simulink model "bess_resource_standalone"  (R2023b)
settings: Solver=ode23t  StartTime=0.0  StopTime=0.8  MaxStep=1e-5  RelTol=1e-3
InitFcn:
  | root=fileparts(fileparts(fileparts(get_param(bdroot,'FileName')))); addpath(root); setup_v2_paths; define_resource_buses(true); define_v2_parameters(true);
undefined symbols (not defined in the file): V2
libraries: ee_lib x12, nesl_utility x9, simulink x3, fl_lib x1
settings Model: Creator=fakebob2004  LastModifiedBy=fakebob2004
settings ModelReferenceCC: UpdateModelReferenceTargets=IfOutOfDate
settings RTWCC: GPUComputeCapability=5.0
settings ConfigComp: CovBoundaryAbsTol=1.0e-5
settings SimscapeCC: SimscapeNominalValues="[{\"value\":\"1\",\"unit\":\"A\"},{\"value\":\"1\",\"unit\":\"bar\"},{\"value\":\"1\",\"unit\":\"cm^2\"},{\"value\":\"1\",\"unit\":\"cm^3/s\"},{\"value\":\"1\",\"unit\":\"kJ/kg\"},{\"value\":\"1\",\"unit\":\"kW\"},{\"value\":\"1\",\"unit\":\"l\"},{\"value\":\"1\",\"unit\":\"N\"},{\"value\":\"1\",\"unit\":\"N*m\"},{\"value\":\"1\",\"unit\":\"V\"},{\"value\":\"0.001\",\"unit\":\"Wb\"}]"  SimscapeLogType=all  SimscapeLogDataHistory=10000

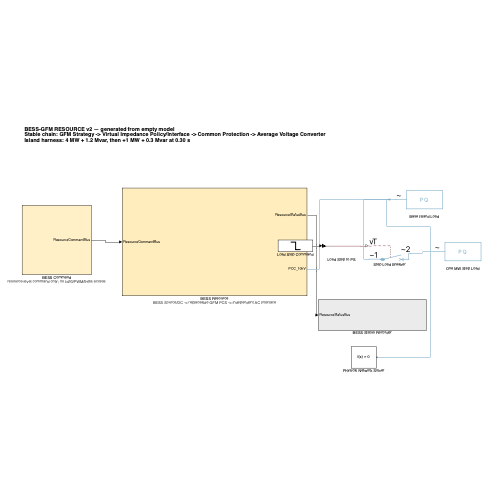
[thumbnail: Simulink's stored preview of the top-level diagram]
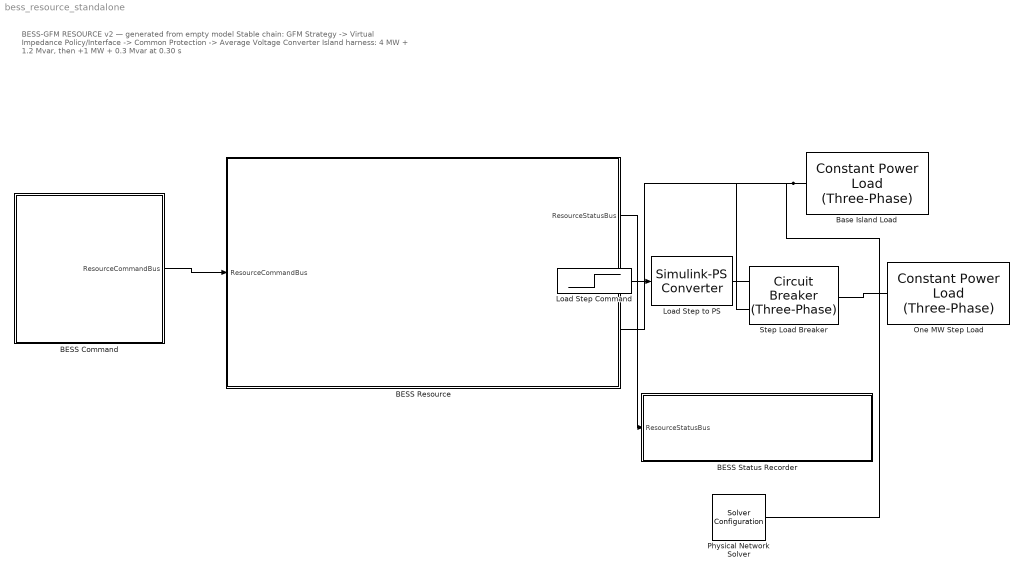
== system bess_resource_standalone ==
  note: BESS-GFM RESOURCE v2 — generated from empty model
      | Stable chain: GFM Strategy -> Virtual Impedance Policy/Interface -> Common Protection -> Average Voltage Converter
      | Island harness: 4 MW + 1.2 Mvar, then +1 MW + 0.3 Mvar at 0.30 s
  BESS Command : Subsystem
      settings: AttributesFormatString=resource-level command only; no Id/Iq/PWM/theta access
  BESS Resource : Subsystem
      settings: AttributesFormatString=BESS Source/DC -> replaceable GFM PCS -> independent AC Interface
  BESS Status Recorder : Subsystem
  Base Island Load : ee_lib/Passive/Constant Power Load (Three-Phase)  port_option=ee.enum.threePhasePort.composite  FRated=V2.BESS.rating.f_Hz Hz  active_power=4e6 W  reactive_power=1.2e6 V*A  Vline_rms_min=0.70*V2.BESS.rating.V_pcc_V V  tau=0.01 s  Vline_rms_ini=V2.BESS.rating.V_pcc_V V  Vang_ini=0 deg  gmin=1e-6 S
  Load Step Command : Step  Time=.30  Before=1  After=0  SampleTime=0
  Load Step to PS : nesl_utility/Simulink-PS Converter  PhysicalDomain=network_engine_domain  SubClassName=ps_input  LeftPortType=input  RightPortType=output  PseudoPeriodic=off  Frequencies=[]  NoiseDistribution=none  NoiseParameters=[]  Unit=V  AffineConversion=off  FilteringAndDerivatives=zero  SimscapeFilterOrder=1  InputFilterTimeConstant=0.001  UdotUserProvided=0
  One MW Step Load : ee_lib/Passive/Constant Power Load (Three-Phase)  port_option=ee.enum.threePhasePort.composite  FRated=V2.BESS.rating.f_Hz Hz  active_power=1e6 W  reactive_power=0.3e6 V*A  Vline_rms_min=0.70*V2.BESS.rating.V_pcc_V V  tau=0.01 s  Vline_rms_ini=V2.BESS.rating.V_pcc_V V  Vang_ini=0 deg  gmin=1e-6 S
  Physical Network Solver : nesl_utility/Solver Configuration  PhysicalDomain=network_engine_domain  SubClassName=solver  LeftPortType=input  RightPortType=generic  Tones=[]  Harmonics=[]  SimulateNoise=off  Profile=off  UseLocalSampling=off  EnableSwitchedLinearOptims=on  FrequencyDomain=off  UseCCode=off  RelTol=0.001  AbsTol=0.001  MinStep=1e-09  ToWorkspace=off  RevertToSquareIcSolve=off  NumHomotopyIterations=100  PhasorMode=off  PhasorModeNumHarmonics=1  ConsistencySolver=NEWTON_XTOL_AFTER_FTOL  CanonicalOrdering=CANONICAL  OptimizeIntermediates=OPTIMIZED  IndexReductionMethod=DerivativeReplacement  DoDC=off  ResidualTolerance=1e-09  ConsistencyTolSource=GLOBAL  ConsistencyAbsTol=0.001  ConsistencyRelTol=0.001  ConsistencyTolFactor=0.001  UseLocalSolver=off  LocalSolverChoice=NE_BACKWARD_EULER_ADVANCER  ResolveIndetEquations=on  FunctionEvalNumThread=1  LocalSolverSampleTime=0.001  DoFixedCost=off  MaxNonlinIter=3  MaxModeIter=2  ComputeImpulses=off  ImpulseIterations=2  LinearAlgebra=auto  LinearAlgebraNumThread=0  EquationFormulation=NE_TIME_EF  DelaysMemoryBudget=1024  AutomaticFiltering=on  FilteringTimeConstant=0.001  PartitionStorageMethod=AS_NEEDED  PartitionMemoryBudget=1024  PartitionMethod=ROBUST  MultibodyUseLocalSolver=off  MultibodyLocalSolverChoice=ODE1  MultibodyLocalSolverSampleTime=0.001
  Step Load Breaker : ee_lib/Switches & Breakers/Circuit Breaker (Three-Phase)  port_option=ee.enum.threePhasePort.composite  control_port_option=ee.enum.controlport.ps  R_closed=0.001 Ohm  G_open=1e-6 1/Ohm  threshold=0.5 V  breaker_behavior=ee.enum.switches.breakerBehavior.zeroCrossingEnable  i_th=1e-8 A
  wires:
  Load Step Command/1 -> Load Step to PS/1
  BESS Command/1(ResourceCommandBus) -> BESS Resource/1(ResourceCommandBus)
  BESS Resource/1(ResourceStatusBus) -> BESS Status Recorder/1(ResourceStatusBus)
  connections:
  Base Island Load/LConn1 -- BESS Resource/RConn1 -- Step Load Breaker/LConn2 -- Physical Network Solver/RConn1
  Step Load Breaker/RConn1 -- One MW Step Load/LConn1
  Load Step to PS/RConn1 -- Step Load Breaker/LConn1

== system bess_resource_standalone/BESS Command ==
  Enable : Constant
  Mode : Constant
  P ref : Constant  Value=4e6
  Q ref : Constant  Value=1.2e6
  Resource Command : BusCreator  Inputs=6  OutDataTypeStr=Bus: ResourceCommandBus
  V ref : Constant  Value=690
  f ref : Constant  Value=50
  ResourceCommandBus : Outport  OutDataTypeStr=Bus: ResourceCommandBus
  wires:
  P ref/1 -> Resource Command/1  "P_ref_W"
  Q ref/1 -> Resource Command/2  "Q_ref_var"
  V ref/1 -> Resource Command/3  "V_ref_V"
  f ref/1 -> Resource Command/4  "f_ref_Hz"
  Enable/1 -> Resource Command/5  "enable"
  Mode/1 -> Resource Command/6  "mode"
  Resource Command/1 -> ResourceCommandBus/1

== system bess_resource_standalone/BESS Resource ==
  ResourceCommandBus : Inport  OutDataTypeStr=Bus: ResourceCommandBus
  01 BESS Source and DC Side : Subsystem
      settings: AttributesFormatString=5 MW / 10 MWh | replaceable energy model -> local limits/status
  02 PCS : Subsystem
      settings: AttributesFormatString=strategy slot -> VI policy/interface -> common protection -> average voltage source
  03 AC Interface : Subsystem
      settings: AttributesFormatString=independent filter + 0.69/10 kV transformer + PCC sensing
  Status Interface : Subsystem
      settings: AttributesFormatString=BESS + GFM PCS + PCC -> ResourceStatusBus
  PCC_10kV : PMIOPort  Side=Right  ConnectionType=Connection: foundation.electrical.three_phase
  ResourceStatusBus : Outport  OutDataTypeStr=Bus: ResourceStatusBus
  wires:
  ResourceCommandBus/1 -> 02 PCS/1(CommandBus)
  03 AC Interface/1(PCCMeasurementBus) -> 01 BESS Source and DC Side/1(PCCMeasurementBus), 02 PCS/2(PCCMeasurementBus), Status Interface/3(PCC)
  01 BESS Source and DC Side/1(BESSStatusBus) -> 02 PCS/3(BESSStatusBus)
  01 BESS Source and DC Side/2(SourceStatusBus) -> Status Interface/1(Source)
  02 PCS/1(GFMPCSStatusBus) -> Status Interface/2(PCS)
  Status Interface/1(ResourceStatusBus) -> ResourceStatusBus/1
  connections:
  02 PCS/RConn1 -- 03 AC Interface/LConn1
  03 AC Interface/RConn1 -- PCC_10kV/RConn1

== system bess_resource_standalone/BESS Status Recorder ==
  ResourceStatusBus : Inport  OutDataTypeStr=Bus: ResourceStatusBus
  BESS v2 Result : ToWorkspace  VariableName=bess_v2_result  SampleTime=-1
  Regression Vector : Mux  Inputs=12
  Status Selector : BusSelector  OutputSignals=P_W,Q_var,Vpcc_V,frequency_Hz,available_power_W,power_headroom_W,current_limit_factor,energy_state_pu,Vdc_V,control_mode,healthy
  Time : Clock
  wires:
  Time/1 -> Regression Vector/1
  Status Selector/1 -> Regression Vector/2  "<P_W>"
  Status Selector/2 -> Regression Vector/3  "<Q_var>"
  Status Selector/3 -> Regression Vector/4  "<Vpcc_V>"
  Status Selector/4 -> Regression Vector/5  "<frequency_Hz>"
  Status Selector/5 -> Regression Vector/6  "<available_power_W>"
  Status Selector/6 -> Regression Vector/7  "<power_headroom_W>"
  Status Selector/7 -> Regression Vector/8  "<current_limit_factor>"
  Status Selector/8 -> Regression Vector/9  "<energy_state_pu>"
  Status Selector/9 -> Regression Vector/10  "<Vdc_V>"
  Status Selector/10 -> Regression Vector/11  "<control_mode>"
  Status Selector/11 -> Regression Vector/12  "<healthy>"
  ResourceStatusBus/1 -> Status Selector/1
  Regression Vector/1 -> BESS v2 Result/1

== system bess_resource_standalone/BESS Resource/01 BESS Source and DC Side ==
  PCCMeasurementBus : Inport  OutDataTypeStr=Bus: PCCMeasurementBus
  01 Energy and DC State : Subsystem
      settings: AttributesFormatString=PCC P -> DC buffer/loss -> SOC, Vdc, Ibat
  02 Limits and Availability : Subsystem
      settings: AttributesFormatString=SOC direction + Ibat limit -> common resource status
  BESSStatusBus : Outport  OutDataTypeStr=Bus: BESSStatusBus
  SourceStatusBus : Outport  Port=2  OutDataTypeStr=Bus: SourceStatusBus
  wires:
  PCCMeasurementBus/1 -> 01 Energy and DC State/1(PCCMeasurementBus)
  01 Energy and DC State/1(BESSDCStateBus) -> 02 Limits and Availability/1(BESSDCStateBus)
  02 Limits and Availability/1(BESSStatusBus) -> BESSStatusBus/1
  02 Limits and Availability/2(SourceStatusBus) -> SourceStatusBus/1

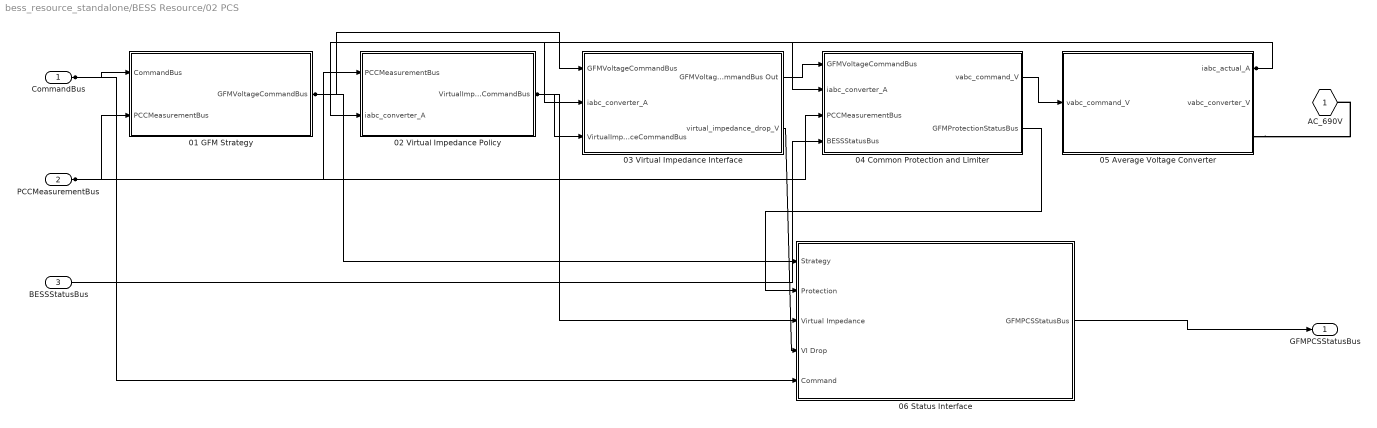
== system bess_resource_standalone/BESS Resource/02 PCS ==
  CommandBus : Inport  OutDataTypeStr=Bus: ResourceCommandBus
  PCCMeasurementBus : Inport  Port=2  OutDataTypeStr=Bus: PCCMeasurementBus
  BESSStatusBus : Inport  Port=3  OutDataTypeStr=Bus: BESSStatusBus
  01 GFM Strategy : Subsystem
      settings: AttributesFormatString=replaceable P-f/Q-V strategy -> typed voltage command
  02 Virtual Impedance Policy : Subsystem
      settings: AttributesFormatString=replaceable static/dynamic VI policy -> enable, R, X
  03 Virtual Impedance Interface : Subsystem
      settings: AttributesFormatString=current conditioning -> R+jX drop -> compensated voltage command
  04 Common Protection and Limiter : Subsystem
      settings: AttributesFormatString=strategy-independent voltage/SOC/current backup protection
  05 Average Voltage Converter : Subsystem
  06 Status Interface : Subsystem
      settings: AttributesFormatString=strategy + VI + protection -> GFMPCSStatusBus
  AC_690V : PMIOPort  Side=Right  ConnectionType=Connection: foundation.electrical.three_phase
  GFMPCSStatusBus : Outport  OutDataTypeStr=Bus: GFMPCSStatusBus
  wires:
  CommandBus/1 -> 01 GFM Strategy/1(CommandBus), 06 Status Interface/5(Command)
  PCCMeasurementBus/1 -> 01 GFM Strategy/2(PCCMeasurementBus), 02 Virtual Impedance Policy/1(PCCMeasurementBus), 04 Common Protection and Limiter/3(PCCMeasurementBus)
  05 Average Voltage Converter/1(iabc_actual_A) -> 02 Virtual Impedance Policy/2(iabc_converter_A), 03 Virtual Impedance Interface/2(iabc_converter_A), 04 Common Protection and Limiter/2(iabc_converter_A)
  01 GFM Strategy/1(GFMVoltageCommandBus) -> 03 Virtual Impedance Interface/1(GFMVoltageCommandBus), 06 Status Interface/1(Strategy)
  02 Virtual Impedance Policy/1(VirtualImpedanceCommandBus) -> 03 Virtual Impedance Interface/3(VirtualImpedanceCommandBus), 06 Status Interface/3(Virtual Impedance)
  03 Virtual Impedance Interface/1(GFMVoltageCommandBus Out) -> 04 Common Protection and Limiter/1(GFMVoltageCommandBus)
  BESSStatusBus/1 -> 04 Common Protection and Limiter/4(BESSStatusBus)
  04 Common Protection and Limiter/1(vabc_command_V) -> 05 Average Voltage Converter/1(vabc_command_V)
  04 Common Protection and Limiter/2(GFMProtectionStatusBus) -> 06 Status Interface/2(Protection)
  03 Virtual Impedance Interface/2(virtual_impedance_drop_V) -> 06 Status Interface/4(VI Drop)
  06 Status Interface/1(GFMPCSStatusBus) -> GFMPCSStatusBus/1
  connections:
  05 Average Voltage Converter/RConn1 -- AC_690V/RConn1

== system bess_resource_standalone/BESS Resource/03 AC Interface ==
  Damped Shunt C : ee_lib/Passive/RLC Assemblies/RLC (Three-Phase)  port_option=ee.enum.threePhasePort.composite  component_structure=ee.enum.rlc.structure.SeriesRC  R=V2.BESS.filter.Rd_ohm Ohm  L=1e-3 H  C=V2.BESS.filter.C_F F  R_parasitic=0 Ohm  G_parasitic=0 1/Ohm  IL_specify=off  IL_priority=High  IL=[0, 0, 0] A  IL_nominal_specify=off  IL_nominal_value=1  IL_nominal_unit=A  VC_specify=off  VC_priority=High  VC=[0, 0, 0] V  VC_nominal_specify=off  VC_nominal_value=1  VC_nominal_unit=V
  Filter Ground : ee_lib/Connectors & References/Grounded Neutral (Three-Phase)  port_option=ee.enum.threePhasePort.composite
  Grid-side R2 + L2 : ee_lib/Passive/RLC Assemblies/RLC (Three-Phase)  port_option=ee.enum.threePhasePort.composite  component_structure=ee.enum.rlc.structure.SeriesRL  R=V2.BESS.filter.R2_ohm Ohm  L=V2.BESS.filter.L2_H H  C=1e-6 F  R_parasitic=0 Ohm  G_parasitic=0 1/Ohm  IL_specify=off  IL_priority=High  IL=[0, 0, 0] A  IL_nominal_specify=off  IL_nominal_value=1  IL_nominal_unit=A  VC_specify=off  VC_priority=High  VC=[0, 0, 0] V  VC_nominal_specify=off  VC_nominal_value=1  VC_nominal_unit=V
  Inverter-side R1 + L1 : ee_lib/Passive/RLC Assemblies/RLC (Three-Phase)  port_option=ee.enum.threePhasePort.composite  component_structure=ee.enum.rlc.structure.SeriesRL  R=V2.BESS.filter.R1_ohm Ohm  L=V2.BESS.filter.L1_H H  C=1e-6 F  R_parasitic=0 Ohm  G_parasitic=0 1/Ohm  IL_specify=off  IL_priority=High  IL=[0, 0, 0] A  IL_nominal_specify=off  IL_nominal_value=1  IL_nominal_unit=A  VC_specify=off  VC_priority=High  VC=[0, 0, 0] V  VC_nominal_specify=off  VC_nominal_value=1  VC_nominal_unit=V
  PCC Measurement : Subsystem
  Step-up Transformer : ee_lib/Passive/Transformers/Two-Winding Transformer (Three-Phase)  SRated=V2.BESS.transformer.S_VA A*V  FRated=V2.BESS.rating.f_Hz Hz  Winding1Connection=ee.enum.windingconnection.Yg  VRated1=V2.BESS.transformer.V1_V V  Winding2Connection=ee.enum.windingconnection.Yg  VRated2=V2.BESS.transformer.V2_V V  CoreType=ee.enum.coretype.threelimb  pu_Rw1=V2.BESS.transformer.R_pu/2  pu_Rw2=V2.BESS.transformer.R_pu/2  leakage_reactance_option=ee.enum.transformer_leakage.exclude  pu_Xl1=0.05  pu_Xl2=0.05  magnetizing_resistance_option=ee.enum.transformer_magnetizingResistance.exclude  pu_Rm=500  magnetizing_reactance_option=ee.enum.transformer_magnetizingReactance.exclude  saturation_option=ee.enum.transformer_saturation.exclude  pu_Xm=500  current_data=[0, .002, 1, 2]  magnetic_flux_data=[0, 1.2, 1.5, 1.51]  pu_X0=0.5  i1_specify=off  i1_priority=None  i1=[0, 0, 0] A  i1_nominal_specify=off  i1_nominal_value=1  i1_nominal_unit=A  i2_specify=off  i2_priority=None  i2=[0, 0, 0] A  i2_nominal_specify=off  i2_nominal_value=1  i2_nominal_unit=A  phi_specify=off  phi_priority=None  phi=[0, 0, 0]  phi_nominal_specify=off  phi_nominal_value=1  phi_nominal_unit=1
  PCS AC Terminal : PMIOPort  Side=Left  ConnectionType=Connection: foundation.electrical.three_phase
  PCC_10kV : PMIOPort  Port=2  Side=Right  ConnectionType=Connection: foundation.electrical.three_phase
  PCCMeasurementBus : Outport  OutDataTypeStr=Bus: PCCMeasurementBus
  wires:
  PCC Measurement/1(PCCMeasurementBus) -> PCCMeasurementBus/1
  connections:
  PCS AC Terminal/RConn1 -- Inverter-side R1 + L1/LConn1
  Grid-side R2 + L2/LConn1 -- Inverter-side R1 + L1/RConn1 -- Damped Shunt C/LConn1
  Damped Shunt C/RConn1 -- Filter Ground/LConn1
  Grid-side R2 + L2/RConn1 -- Step-up Transformer/LConn1
  Step-up Transformer/RConn1 -- PCC Measurement/LConn1
  PCC Measurement/RConn1 -- PCC_10kV/RConn1

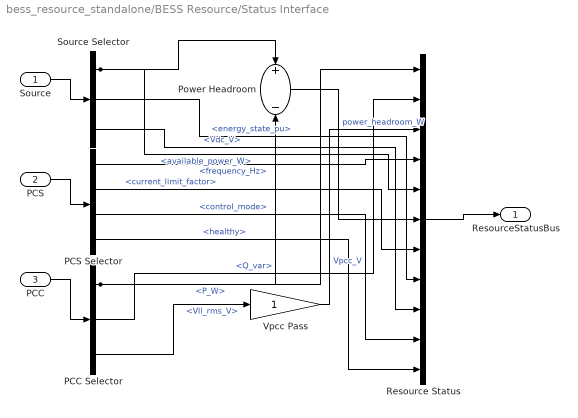
== system bess_resource_standalone/BESS Resource/Status Interface ==
  Source : Inport  OutDataTypeStr=Bus: SourceStatusBus
  PCS : Inport  Port=2  OutDataTypeStr=Bus: GFMPCSStatusBus
  PCC : Inport  Port=3  OutDataTypeStr=Bus: PCCMeasurementBus
  PCC Selector : BusSelector  OutputSignals=P_W,Q_var,Vll_rms_V
  PCS Selector : BusSelector  OutputSignals=frequency_Hz,current_limit_factor,control_mode,healthy
  Power Headroom : Sum  Inputs=+-
  Resource Status : BusCreator  Inputs=11  OutDataTypeStr=Bus: ResourceStatusBus
  Source Selector : BusSelector  OutputSignals=available_power_W,energy_state_pu,Vdc_V
  Vpcc Pass : Gain
  ResourceStatusBus : Outport  OutDataTypeStr=Bus: ResourceStatusBus
  wires:
  Source/1 -> Source Selector/1
  PCS/1 -> PCS Selector/1
  PCC/1 -> PCC Selector/1
  Source Selector/1 -> Power Headroom/1, Resource Status/5  "<available_power_W>"
  PCC Selector/1 -> Power Headroom/2, Resource Status/1  "<P_W>"
  PCC Selector/3 -> Vpcc Pass/1  "<Vll_rms_V>"
  PCC Selector/2 -> Resource Status/2  "<Q_var>"
  Vpcc Pass/1 -> Resource Status/3  "Vpcc_V"
  PCS Selector/1 -> Resource Status/4  "<frequency_Hz>"
  Power Headroom/1 -> Resource Status/6  "power_headroom_W"
  PCS Selector/2 -> Resource Status/7  "<current_limit_factor>"
  Source Selector/2 -> Resource Status/8  "<energy_state_pu>"
  Source Selector/3 -> Resource Status/9  "<Vdc_V>"
  PCS Selector/3 -> Resource Status/10  "<control_mode>"
  PCS Selector/4 -> Resource Status/11  "<healthy>"
  Resource Status/1 -> ResourceStatusBus/1

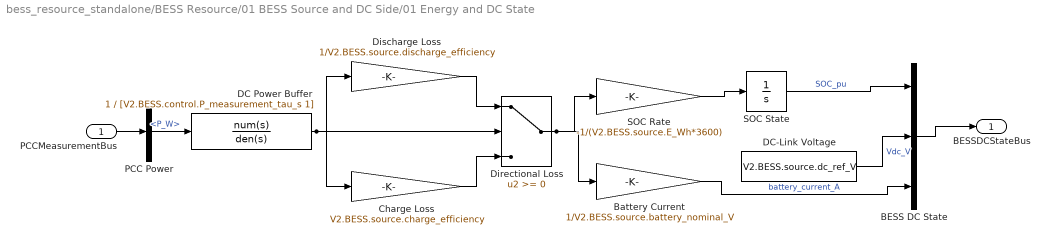
== system bess_resource_standalone/BESS Resource/01 BESS Source and DC Side/01 Energy and DC State ==
  PCCMeasurementBus : Inport  OutDataTypeStr=Bus: PCCMeasurementBus
  BESS DC State : BusCreator  Inputs=3  OutDataTypeStr=Bus: BESSDCStateBus
  Battery Current : Gain  Gain=1/V2.BESS.source.battery_nominal_V
  Charge Loss : Gain  Gain=V2.BESS.source.charge_efficiency
  DC Power Buffer : TransferFcn  Numerator=1  Denominator=[V2.BESS.control.P_measurement_tau_s 1]
  DC-Link Voltage : Constant  Value=V2.BESS.source.dc_ref_V
  Directional Loss : Switch  SaturateOnIntegerOverflow=off  InputSameDT=off
  Discharge Loss : Gain  Gain=1/V2.BESS.source.discharge_efficiency
  PCC Power : BusSelector  OutputSignals=P_W
  SOC Rate : Gain  Gain=-1/(V2.BESS.source.E_Wh*3600)
  SOC State : Integrator  InitialCondition=V2.BESS.source.SOC_initial  LimitOutput=on  UpperSaturationLimit=V2.BESS.source.SOC_max  LowerSaturationLimit=V2.BESS.source.SOC_min
  BESSDCStateBus : Outport  OutDataTypeStr=Bus: BESSDCStateBus
  wires:
  PCCMeasurementBus/1 -> PCC Power/1
  PCC Power/1 -> DC Power Buffer/1  "<P_W>"
  DC Power Buffer/1 -> Discharge Loss/1, Directional Loss/2, Charge Loss/1
  Discharge Loss/1 -> Directional Loss/1
  Charge Loss/1 -> Directional Loss/3
  Directional Loss/1 -> SOC Rate/1, Battery Current/1
  SOC Rate/1 -> SOC State/1
  SOC State/1 -> BESS DC State/1  "SOC_pu"
  DC-Link Voltage/1 -> BESS DC State/2  "Vdc_V"
  Battery Current/1 -> BESS DC State/3  "battery_current_A"
  BESS DC State/1 -> BESSDCStateBus/1

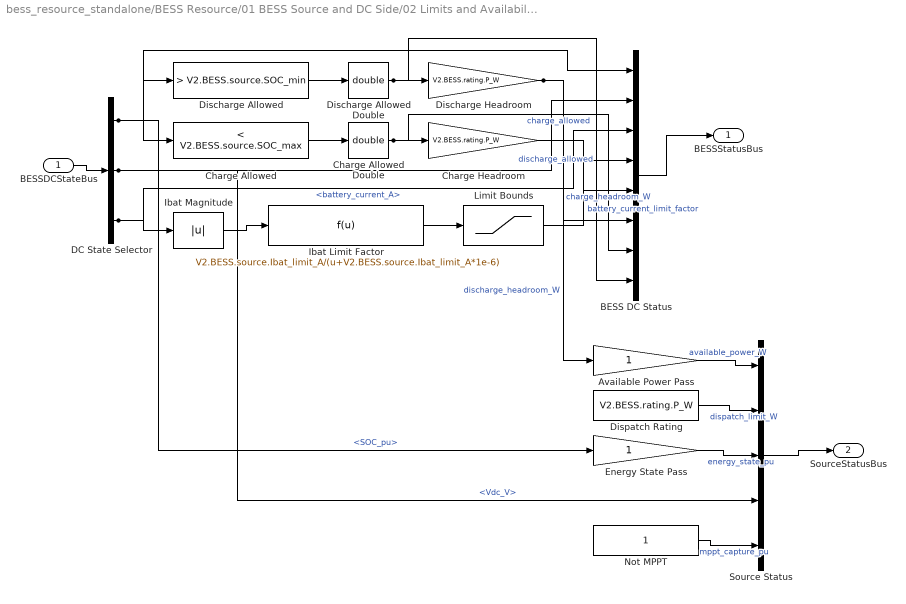
== system bess_resource_standalone/BESS Resource/01 BESS Source and DC Side/02 Limits and Availability ==
  BESSDCStateBus : Inport  OutDataTypeStr=Bus: BESSDCStateBus
  Available Power Pass : Gain
  BESS DC Status : BusCreator  Inputs=8  OutDataTypeStr=Bus: BESSStatusBus
  Charge Allowed : simulink/Logic and Bit Operations/Compare To Constant  relop=<  const=V2.BESS.source.SOC_max  OutDataTypeStr=boolean
  Charge Allowed Double : DataTypeConversion  OutDataTypeStr=double  SaturateOnIntegerOverflow=off  RndMeth=Floor
  Charge Headroom : Gain  Gain=V2.BESS.rating.P_W
  DC State Selector : BusSelector  OutputSignals=SOC_pu,Vdc_V,battery_current_A
  Discharge Allowed : simulink/Logic and Bit Operations/Compare To Constant  relop=>  const=V2.BESS.source.SOC_min  OutDataTypeStr=boolean
  Discharge Allowed Double : DataTypeConversion  OutDataTypeStr=double  SaturateOnIntegerOverflow=off  RndMeth=Floor
  Discharge Headroom : Gain  Gain=V2.BESS.rating.P_W
  Dispatch Rating : Constant  Value=V2.BESS.rating.P_W
  Energy State Pass : Gain
  Ibat Limit Factor : Fcn  Expr=V2.BESS.source.Ibat_limit_A/(u+V2.BESS.source.Ibat_limit_A*1e-6)
  Ibat Magnitude : Abs  SaturateOnIntegerOverflow=off
  Limit Bounds : Saturate  UpperLimit=1  LowerLimit=0
  Not MPPT : Constant
  Source Status : BusCreator  Inputs=5  OutDataTypeStr=Bus: SourceStatusBus
  BESSStatusBus : Outport  OutDataTypeStr=Bus: BESSStatusBus
  SourceStatusBus : Outport  Port=2  OutDataTypeStr=Bus: SourceStatusBus
  wires:
  BESSDCStateBus/1 -> DC State Selector/1
  DC State Selector/1 -> Discharge Allowed/1, Charge Allowed/1, BESS DC Status/1, Energy State Pass/1  "<SOC_pu>"
  DC State Selector/3 -> Ibat Magnitude/1, BESS DC Status/3  "<battery_current_A>"
  Ibat Magnitude/1 -> Ibat Limit Factor/1
  Ibat Limit Factor/1 -> Limit Bounds/1
  Discharge Allowed/1 -> Discharge Allowed Double/1
  Charge Allowed/1 -> Charge Allowed Double/1
  Discharge Allowed Double/1 -> Discharge Headroom/1, BESS DC Status/8  "discharge_allowed"
  Charge Allowed Double/1 -> Charge Headroom/1, BESS DC Status/7  "charge_allowed"
  DC State Selector/2 -> BESS DC Status/2, Source Status/4  "<Vdc_V>"
  Limit Bounds/1 -> BESS DC Status/4  "battery_current_limit_factor"
  Charge Headroom/1 -> BESS DC Status/5  "charge_headroom_W"
  Discharge Headroom/1 -> BESS DC Status/6, Available Power Pass/1  "discharge_headroom_W"
  BESS DC Status/1 -> BESSStatusBus/1
  Available Power Pass/1 -> Source Status/1  "available_power_W"
  Dispatch Rating/1 -> Source Status/2  "dispatch_limit_W"
  Energy State Pass/1 -> Source Status/3  "energy_state_pu"
  Not MPPT/1 -> Source Status/5  "mppt_capture_pu"
  Source Status/1 -> SourceStatusBus/1

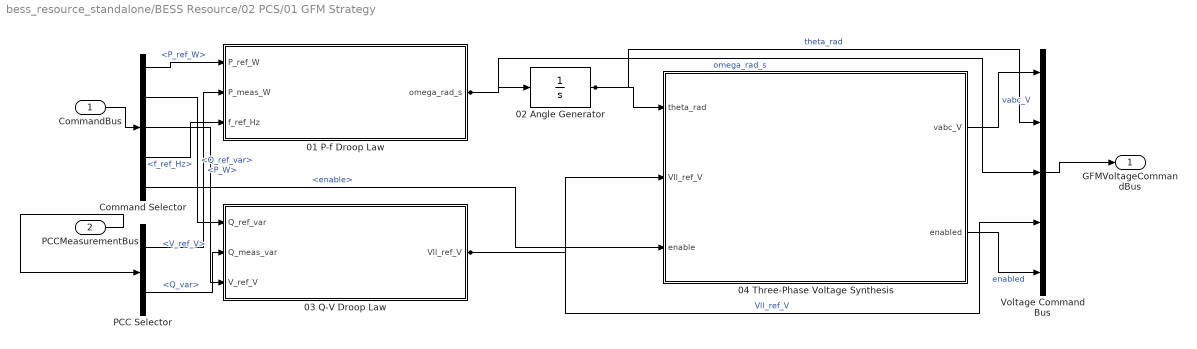
== system bess_resource_standalone/BESS Resource/02 PCS/01 GFM Strategy ==
  CommandBus : Inport  OutDataTypeStr=Bus: ResourceCommandBus
  PCCMeasurementBus : Inport  Port=2  OutDataTypeStr=Bus: PCCMeasurementBus
  01 P-f Droop Law : Subsystem
      settings: AttributesFormatString=omega = 2*pi*fref + mp*(Pref-P)
  02 Angle Generator : Integrator  InitialCondition=V2.BESS.control.theta0_rad
  03 Q-V Droop Law : Subsystem
      settings: AttributesFormatString=Vll = Vref + nq*(Qref-Q)
  04 Three-Phase Voltage Synthesis : Subsystem
      settings: AttributesFormatString=theta + Vll + enable -> vabc
  Command Selector : BusSelector  OutputSignals=P_ref_W,Q_ref_var,V_ref_V,f_ref_Hz,enable
  PCC Selector : BusSelector  OutputSignals=P_W,Q_var
  Voltage Command Bus : BusCreator  Inputs=5  OutDataTypeStr=Bus: GFMVoltageCommandBus
  GFMVoltageCommandBus : Outport  OutDataTypeStr=Bus: GFMVoltageCommandBus
  wires:
  CommandBus/1 -> Command Selector/1
  PCCMeasurementBus/1 -> PCC Selector/1
  Command Selector/1 -> 01 P-f Droop Law/1(P_ref_W)  "<P_ref_W>"
  PCC Selector/1 -> 01 P-f Droop Law/2(P_meas_W)  "<P_W>"
  Command Selector/4 -> 01 P-f Droop Law/3(f_ref_Hz)  "<f_ref_Hz>"
  01 P-f Droop Law/1(omega_rad_s) -> 02 Angle Generator/1, Voltage Command Bus/3  "omega_rad_s"
  Command Selector/2 -> 03 Q-V Droop Law/1(Q_ref_var)  "<Q_ref_var>"
  PCC Selector/2 -> 03 Q-V Droop Law/2(Q_meas_var)  "<Q_var>"
  Command Selector/3 -> 03 Q-V Droop Law/3(V_ref_V)  "<V_ref_V>"
  02 Angle Generator/1 -> 04 Three-Phase Voltage Synthesis/1(theta_rad), Voltage Command Bus/2  "theta_rad"
  03 Q-V Droop Law/1(Vll_ref_V) -> 04 Three-Phase Voltage Synthesis/2(Vll_ref_V), Voltage Command Bus/4  "Vll_ref_V"
  Command Selector/5 -> 04 Three-Phase Voltage Synthesis/3(enable)  "<enable>"
  04 Three-Phase Voltage Synthesis/1(vabc_V) -> Voltage Command Bus/1  "vabc_V"
  04 Three-Phase Voltage Synthesis/2(enabled) -> Voltage Command Bus/5  "enabled"
  Voltage Command Bus/1 -> GFMVoltageCommandBus/1

== system bess_resource_standalone/BESS Resource/02 PCS/02 Virtual Impedance Policy ==
  PCCMeasurementBus : Inport  OutDataTypeStr=Bus: PCCMeasurementBus
  iabc_converter_A : Inport  Port=2
  R virtual : Constant  Value=V2.BESS.control.Rvirt_pu*(V2.BESS.rating.V_ac_low_V^2/V2.BESS.rating.S_VA)
  Reserved Current Input : Terminator
  Reserved PCC Input : Terminator
  VI Command : BusCreator  Inputs=3  OutDataTypeStr=Bus: VirtualImpedanceCommandBus
  VI Enable : Constant  Value=V2.BESS.control.virtual_impedance_enabled
  X virtual : Constant  Value=V2.BESS.control.Xvirt_pu*(V2.BESS.rating.V_ac_low_V^2/V2.BESS.rating.S_VA)
  VirtualImpedanceCommandBus : Outport  OutDataTypeStr=Bus: VirtualImpedanceCommandBus
  wires:
  PCCMeasurementBus/1 -> Reserved PCC Input/1
  iabc_converter_A/1 -> Reserved Current Input/1
  VI Enable/1 -> VI Command/1  "enable"
  R virtual/1 -> VI Command/2  "R_ohm"
  X virtual/1 -> VI Command/3  "X_ohm"
  VI Command/1 -> VirtualImpedanceCommandBus/1

== system bess_resource_standalone/BESS Resource/02 PCS/03 Virtual Impedance Interface ==
  GFMVoltageCommandBus : Inport  OutDataTypeStr=Bus: GFMVoltageCommandBus
  iabc_converter_A : Inport  Port=2
  VirtualImpedanceCommandBus : Inport  Port=3  OutDataTypeStr=Bus: VirtualImpedanceCommandBus
  01 Current Conditioning : Subsystem
      settings: AttributesFormatString=abc measurement filters + Clarke transform
  02 R+jX Drop : Subsystem
      settings: AttributesFormatString=dV = enable*(R*i + X*J*i)
  03 Voltage Command Compensation : Subsystem
      settings: AttributesFormatString=raw voltage command - virtual drop
  GFMVoltageCommandBus Out : Outport  OutDataTypeStr=Bus: GFMVoltageCommandBus
  virtual_impedance_drop_V : Outport  Port=2
  wires:
  iabc_converter_A/1 -> 01 Current Conditioning/1(iabc_A)
  01 Current Conditioning/1(i_alpha_beta_A) -> 02 R+jX Drop/1(i_alpha_beta_A)
  VirtualImpedanceCommandBus/1 -> 02 R+jX Drop/2(VirtualImpedanceCommandBus)
  GFMVoltageCommandBus/1 -> 03 Voltage Command Compensation/1(GFMVoltageCommandBus)
  02 R+jX Drop/1(dVabc_V) -> 03 Voltage Command Compensation/2(dVabc_V)
  03 Voltage Command Compensation/1(GFMVoltageCommandBus Out) -> GFMVoltageCommandBus Out/1
  02 R+jX Drop/2(drop_rms_V) -> virtual_impedance_drop_V/1

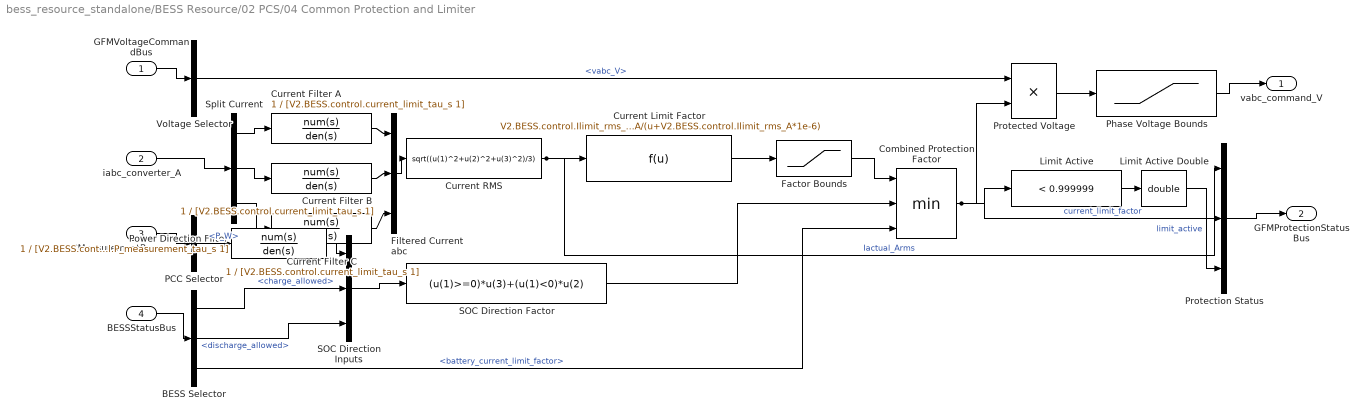
== system bess_resource_standalone/BESS Resource/02 PCS/04 Common Protection and Limiter ==
  GFMVoltageCommandBus : Inport  OutDataTypeStr=Bus: GFMVoltageCommandBus
  iabc_converter_A : Inport  Port=2
  PCCMeasurementBus : Inport  Port=3  OutDataTypeStr=Bus: PCCMeasurementBus
  BESSStatusBus : Inport  Port=4  OutDataTypeStr=Bus: BESSStatusBus
  BESS Selector : BusSelector  OutputSignals=charge_allowed,discharge_allowed,battery_current_limit_factor
  Combined Protection Factor : MinMax  Inputs=3
  Current Filter A : TransferFcn  Numerator=1  Denominator=[V2.BESS.control.current_limit_tau_s 1]
  Current Filter B : TransferFcn  Numerator=1  Denominator=[V2.BESS.control.current_limit_tau_s 1]
  Current Filter C : TransferFcn  Numerator=1  Denominator=[V2.BESS.control.current_limit_tau_s 1]
  Current Limit Factor : Fcn  Expr=V2.BESS.control.Ilimit_rms_A/(u+V2.BESS.control.Ilimit_rms_A*1e-6)
  Current RMS : Fcn  Expr=sqrt((u(1)^2+u(2)^2+u(3)^2)/3)
  Factor Bounds : Saturate  UpperLimit=1  LowerLimit=0
  Filtered Current abc : Mux  Inputs=3
  Limit Active : simulink/Logic and Bit Operations/Compare To Constant  relop=<  const=0.999999  OutDataTypeStr=boolean
  Limit Active Double : DataTypeConversion  OutDataTypeStr=double  SaturateOnIntegerOverflow=off  RndMeth=Floor
  PCC Selector : BusSelector  OutputSignals=P_W
  Phase Voltage Bounds : Saturate  UpperLimit=sqrt(2/3)*V2.BESS.control.Vmax_pu*V2.BESS.rating.V_ac_low_V  LowerLimit=-sqrt(2/3)*V2.BESS.control.Vmax_pu*V2.BESS.rating.V_ac_low_V
  Power Direction Filter : TransferFcn  Numerator=1  Denominator=[V2.BESS.control.P_measurement_tau_s 1]
  Protected Voltage : Product
  Protection Status : BusCreator  Inputs=3  OutDataTypeStr=Bus: GFMProtectionStatusBus
  SOC Direction Factor : Fcn  Expr=(u(1)>=0)*u(3)+(u(1)<0)*u(2)
  SOC Direction Inputs : Mux  Inputs=3
  Split Current : Demux  Outputs=3
  Voltage Selector : BusSelector  OutputSignals=vabc_V
  vabc_command_V : Outport
  GFMProtectionStatusBus : Outport  Port=2  OutDataTypeStr=Bus: GFMProtectionStatusBus
  wires:
  GFMVoltageCommandBus/1 -> Voltage Selector/1
  PCCMeasurementBus/1 -> PCC Selector/1
  BESSStatusBus/1 -> BESS Selector/1
  iabc_converter_A/1 -> Split Current/1
  Split Current/1 -> Current Filter A/1
  Current Filter A/1 -> Filtered Current abc/1
  Split Current/2 -> Current Filter B/1
  Current Filter B/1 -> Filtered Current abc/2
  Split Current/3 -> Current Filter C/1
  Current Filter C/1 -> Filtered Current abc/3
  Filtered Current abc/1 -> Current RMS/1
  Current RMS/1 -> Current Limit Factor/1, Protection Status/1  "Iactual_Arms"
  Current Limit Factor/1 -> Factor Bounds/1
  PCC Selector/1 -> Power Direction Filter/1  "<P_W>"
  Power Direction Filter/1 -> SOC Direction Inputs/1
  BESS Selector/1 -> SOC Direction Inputs/2  "<charge_allowed>"
  BESS Selector/2 -> SOC Direction Inputs/3  "<discharge_allowed>"
  SOC Direction Inputs/1 -> SOC Direction Factor/1
  Factor Bounds/1 -> Combined Protection Factor/1
  SOC Direction Factor/1 -> Combined Protection Factor/2
  BESS Selector/3 -> Combined Protection Factor/3  "<battery_current_limit_factor>"
  Voltage Selector/1 -> Protected Voltage/1  "<vabc_V>"
  Combined Protection Factor/1 -> Protected Voltage/2, Limit Active/1, Protection Status/2  "current_limit_factor"
  Protected Voltage/1 -> Phase Voltage Bounds/1
  Limit Active/1 -> Limit Active Double/1
  Phase Voltage Bounds/1 -> vabc_command_V/1
  Limit Active Double/1 -> Protection Status/3  "limit_active"
  Protection Status/1 -> GFMProtectionStatusBus/1

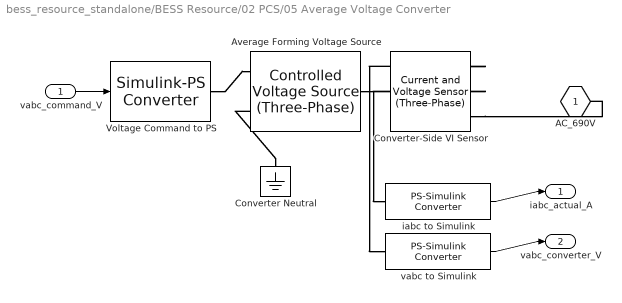
== system bess_resource_standalone/BESS Resource/02 PCS/05 Average Voltage Converter ==
  vabc_command_V : Inport
  Average Forming Voltage Source : ee_lib/Sources/Controlled Voltage Source (Three-Phase)  input_option=ee.enum.inputType.instantaneous  FRated=V2.BESS.rating.f_Hz Hz
  Converter Neutral : fl_lib/Electrical/Electrical Elements/Electrical Reference
  Converter-Side VI Sensor : ee_lib/Sensors & Transducers/Current and Voltage Sensor (Three-Phase)  port_option=ee.enum.threePhasePort.composite  vMeasurementType=ee.enum.vmeasurement.ll  outputUnit=ee.enum.unit.si  SRated=100e6 A*V  VRated=24e3 V  I_specify=off  I_priority=None  I=[0, 0, 0] A  I_nominal_specify=off  I_nominal_value=1  I_nominal_unit=A  V_specify=off  V_priority=None  V=[0, 0, 0] V  V_nominal_specify=off  V_nominal_value=1  V_nominal_unit=V
  Voltage Command to PS : nesl_utility/Simulink-PS Converter  PhysicalDomain=network_engine_domain  SubClassName=ps_input  LeftPortType=input  RightPortType=output  PseudoPeriodic=off  Frequencies=[]  NoiseDistribution=none  NoiseParameters=[]  Unit=V  AffineConversion=off  FilteringAndDerivatives=zero  SimscapeFilterOrder=1  InputFilterTimeConstant=0.001  UdotUserProvided=0
  iabc to Simulink : nesl_utility/PS-Simulink Converter  PhysicalDomain=network_engine_domain  SubClassName=ps_output  LeftPortType=input  RightPortType=output  PseudoPeriodic=off  Frequencies=[]  VectorFormat=inherit  Unit=A  AffineConversion=off
  vabc to Simulink : nesl_utility/PS-Simulink Converter  PhysicalDomain=network_engine_domain  SubClassName=ps_output  LeftPortType=input  RightPortType=output  PseudoPeriodic=off  Frequencies=[]  VectorFormat=inherit  Unit=V  AffineConversion=off
  AC_690V : PMIOPort  Side=Right  ConnectionType=Connection: foundation.electrical.three_phase
  iabc_actual_A : Outport
  vabc_converter_V : Outport  Port=2
  wires:
  vabc_command_V/1 -> Voltage Command to PS/1
  iabc to Simulink/1 -> iabc_actual_A/1
  vabc to Simulink/1 -> vabc_converter_V/1
  connections:
  Voltage Command to PS/RConn1 -- Average Forming Voltage Source/LConn1
  Average Forming Voltage Source/LConn2 -- Converter Neutral/LConn1
  Average Forming Voltage Source/RConn1 -- Converter-Side VI Sensor/LConn1
  Converter-Side VI Sensor/RConn3 -- AC_690V/RConn1
  Converter-Side VI Sensor/RConn2 -- iabc to Simulink/LConn1
  Converter-Side VI Sensor/RConn1 -- vabc to Simulink/LConn1

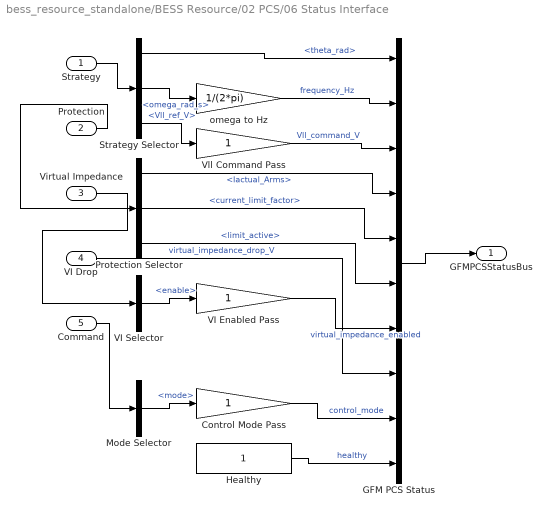
== system bess_resource_standalone/BESS Resource/02 PCS/06 Status Interface ==
  Strategy : Inport  OutDataTypeStr=Bus: GFMVoltageCommandBus
  Protection : Inport  Port=2  OutDataTypeStr=Bus: GFMProtectionStatusBus
  Virtual Impedance : Inport  Port=3  OutDataTypeStr=Bus: VirtualImpedanceCommandBus
  VI Drop : Inport  Port=4
  Command : Inport  Port=5  OutDataTypeStr=Bus: ResourceCommandBus
  Control Mode Pass : Gain
  GFM PCS Status : BusCreator  Inputs=10  OutDataTypeStr=Bus: GFMPCSStatusBus
  Healthy : Constant
  Mode Selector : BusSelector  OutputSignals=mode
  Protection Selector : BusSelector  OutputSignals=Iactual_Arms,current_limit_factor,limit_active
  Strategy Selector : BusSelector  OutputSignals=theta_rad,omega_rad_s,Vll_ref_V
  VI Enabled Pass : Gain
  VI Selector : BusSelector  OutputSignals=enable
  Vll Command Pass : Gain
  omega to Hz : Gain  Gain=1/(2*pi)
  GFMPCSStatusBus : Outport  OutDataTypeStr=Bus: GFMPCSStatusBus
  wires:
  Strategy/1 -> Strategy Selector/1
  Protection/1 -> Protection Selector/1
  Virtual Impedance/1 -> VI Selector/1
  Command/1 -> Mode Selector/1
  Strategy Selector/2 -> omega to Hz/1  "<omega_rad_s>"
  Strategy Selector/3 -> Vll Command Pass/1  "<Vll_ref_V>"
  VI Selector/1 -> VI Enabled Pass/1  "<enable>"
  Mode Selector/1 -> Control Mode Pass/1  "<mode>"
  Strategy Selector/1 -> GFM PCS Status/1  "<theta_rad>"
  omega to Hz/1 -> GFM PCS Status/2  "frequency_Hz"
  Vll Command Pass/1 -> GFM PCS Status/3  "Vll_command_V"
  Protection Selector/1 -> GFM PCS Status/4  "<Iactual_Arms>"
  Protection Selector/2 -> GFM PCS Status/5  "<current_limit_factor>"
  Protection Selector/3 -> GFM PCS Status/6  "<limit_active>"
  VI Enabled Pass/1 -> GFM PCS Status/7  "virtual_impedance_enabled"
  VI Drop/1 -> GFM PCS Status/8  "virtual_impedance_drop_V"
  Control Mode Pass/1 -> GFM PCS Status/9  "control_mode"
  Healthy/1 -> GFM PCS Status/10  "healthy"
  GFM PCS Status/1 -> GFMPCSStatusBus/1

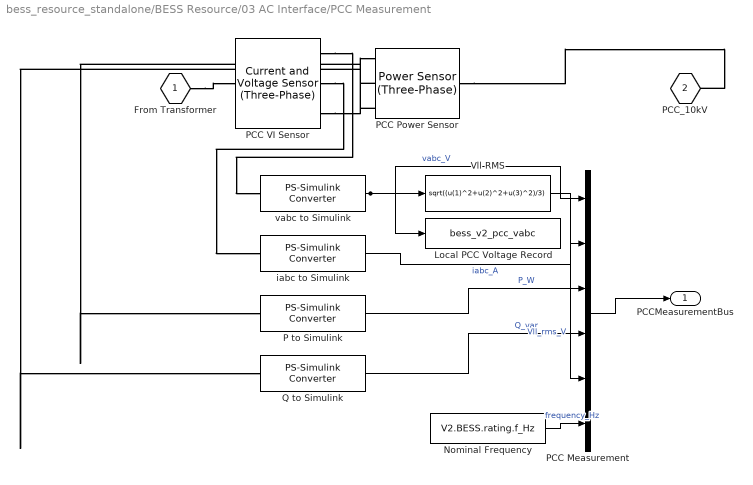
== system bess_resource_standalone/BESS Resource/03 AC Interface/PCC Measurement ==
  Local PCC Voltage Record : ToWorkspace  VariableName=bess_v2_pcc_vabc  SampleTime=-1
  Nominal Frequency : Constant  Value=V2.BESS.rating.f_Hz
  P to Simulink : nesl_utility/PS-Simulink Converter  PhysicalDomain=network_engine_domain  SubClassName=ps_output  LeftPortType=input  RightPortType=output  PseudoPeriodic=off  Frequencies=[]  VectorFormat=inherit  Unit=W  AffineConversion=off
  PCC Measurement : BusCreator  Inputs=6  OutDataTypeStr=Bus: PCCMeasurementBus
  PCC Power Sensor : ee_lib/Sensors & Transducers/Power Sensor (Three-Phase)  port_option=ee.enum.threePhasePort.composite  load_type=ee.enum.passive.type_balanced.balanced  f0=60 Hz
  PCC VI Sensor : ee_lib/Sensors & Transducers/Current and Voltage Sensor (Three-Phase)  port_option=ee.enum.threePhasePort.composite  vMeasurementType=ee.enum.vmeasurement.ll  outputUnit=ee.enum.unit.si  SRated=100e6 A*V  VRated=24e3 V  I_specify=off  I_priority=None  I=[0, 0, 0] A  I_nominal_specify=off  I_nominal_value=1  I_nominal_unit=A  V_specify=off  V_priority=None  V=[0, 0, 0] V  V_nominal_specify=off  V_nominal_value=1  V_nominal_unit=V
  Q to Simulink : nesl_utility/PS-Simulink Converter  PhysicalDomain=network_engine_domain  SubClassName=ps_output  LeftPortType=input  RightPortType=output  PseudoPeriodic=off  Frequencies=[]  VectorFormat=inherit  Unit=W  AffineConversion=off
  Vll RMS : Fcn  Expr=sqrt((u(1)^2+u(2)^2+u(3)^2)/3)
  iabc to Simulink : nesl_utility/PS-Simulink Converter  PhysicalDomain=network_engine_domain  SubClassName=ps_output  LeftPortType=input  RightPortType=output  PseudoPeriodic=off  Frequencies=[]  VectorFormat=inherit  Unit=A  AffineConversion=off
  vabc to Simulink : nesl_utility/PS-Simulink Converter  PhysicalDomain=network_engine_domain  SubClassName=ps_output  LeftPortType=input  RightPortType=output  PseudoPeriodic=off  Frequencies=[]  VectorFormat=inherit  Unit=V  AffineConversion=off
  From Transformer : PMIOPort  Side=Left  ConnectionType=Connection: foundation.electrical.three_phase
  PCC_10kV : PMIOPort  Port=2  Side=Right  ConnectionType=Connection: foundation.electrical.three_phase
  PCCMeasurementBus : Outport  OutDataTypeStr=Bus: PCCMeasurementBus
  wires:
  vabc to Simulink/1 -> Vll RMS/1, Local PCC Voltage Record/1, PCC Measurement/1  "vabc_V"
  iabc to Simulink/1 -> PCC Measurement/2  "iabc_A"
  P to Simulink/1 -> PCC Measurement/3  "P_W"
  Q to Simulink/1 -> PCC Measurement/4  "Q_var"
  Vll RMS/1 -> PCC Measurement/5  "Vll_rms_V"
  Nominal Frequency/1 -> PCC Measurement/6  "frequency_Hz"
  PCC Measurement/1 -> PCCMeasurementBus/1
  connections:
  From Transformer/RConn1 -- PCC VI Sensor/LConn1
  PCC VI Sensor/RConn3 -- PCC Power Sensor/LConn1
  PCC Power Sensor/RConn1 -- PCC_10kV/RConn1
  PCC VI Sensor/RConn1 -- vabc to Simulink/LConn1
  PCC VI Sensor/RConn2 -- iabc to Simulink/LConn1
  PCC Power Sensor/LConn2 -- P to Simulink/LConn1
  PCC Power Sensor/LConn3 -- Q to Simulink/LConn1

== system bess_resource_standalone/BESS Resource/02 PCS/01 GFM Strategy/01 P-f Droop Law ==
  P_ref_W : Inport
  P_meas_W : Inport  Port=2
  f_ref_Hz : Inport  Port=3
  Frequency Reference : Gain  Gain=2*pi
  Omega Command : Sum
  P Error : Sum  Inputs=+-
  P Measurement Filter : TransferFcn  Numerator=1  Denominator=[V2.BESS.control.P_measurement_tau_s 1]
  P-f Droop : Gain  Gain=2*pi*V2.BESS.control.P_f_Hz_per_MW/1e6
  omega_rad_s : Outport
  wires:
  P_ref_W/1 -> P Error/1
  P_meas_W/1 -> P Measurement Filter/1
  P Measurement Filter/1 -> P Error/2
  P Error/1 -> P-f Droop/1
  P-f Droop/1 -> Omega Command/1
  f_ref_Hz/1 -> Frequency Reference/1
  Frequency Reference/1 -> Omega Command/2
  Omega Command/1 -> omega_rad_s/1

== system bess_resource_standalone/BESS Resource/02 PCS/01 GFM Strategy/03 Q-V Droop Law ==
  Q_ref_var : Inport
  Q_meas_var : Inport  Port=2
  V_ref_V : Inport  Port=3
  Q Error : Sum  Inputs=+-
  Q Measurement Filter : TransferFcn  Numerator=1  Denominator=[V2.BESS.control.Q_measurement_tau_s 1]
  Q-V Droop : Gain  Gain=V2.BESS.control.Q_V_V_per_Mvar/1e6
  Voltage Bounds : Saturate  UpperLimit=V2.BESS.control.Vmax_pu*V2.BESS.rating.V_ac_low_V  LowerLimit=V2.BESS.control.Vmin_pu*V2.BESS.rating.V_ac_low_V
  Voltage Command : Sum
  Vll_ref_V : Outport
  wires:
  Q_ref_var/1 -> Q Error/1
  Q_meas_var/1 -> Q Measurement Filter/1
  Q Measurement Filter/1 -> Q Error/2
  Q Error/1 -> Q-V Droop/1
  Q-V Droop/1 -> Voltage Command/1
  V_ref_V/1 -> Voltage Command/2
  Voltage Command/1 -> Voltage Bounds/1
  Voltage Bounds/1 -> Vll_ref_V/1

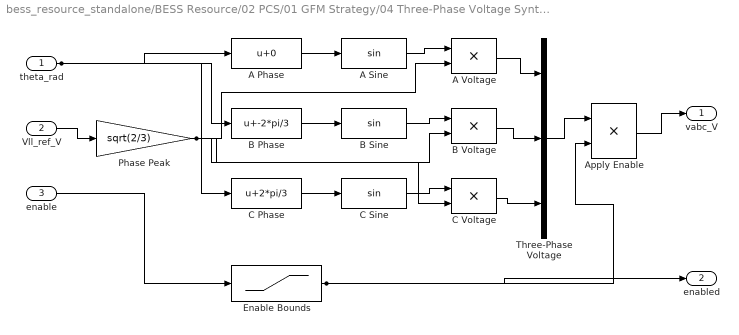
== system bess_resource_standalone/BESS Resource/02 PCS/01 GFM Strategy/04 Three-Phase Voltage Synthesis ==
  theta_rad : Inport
  Vll_ref_V : Inport  Port=2
  enable : Inport  Port=3
  A Phase : Bias  SaturateOnIntegerOverflow=off
  A Sine : Trigonometry
  A Voltage : Product
  Apply Enable : Product
  B Phase : Bias  Bias=-2*pi/3  SaturateOnIntegerOverflow=off
  B Sine : Trigonometry
  B Voltage : Product
  C Phase : Bias  Bias=2*pi/3  SaturateOnIntegerOverflow=off
  C Sine : Trigonometry
  C Voltage : Product
  Enable Bounds : Saturate  UpperLimit=1  LowerLimit=0
  Phase Peak : Gain  Gain=sqrt(2/3)
  Three-Phase Voltage : Mux  Inputs=3
  vabc_V : Outport
  enabled : Outport  Port=2
  wires:
  theta_rad/1 -> A Phase/1, B Phase/1, C Phase/1
  A Phase/1 -> A Sine/1
  A Sine/1 -> A Voltage/1
  Phase Peak/1 -> A Voltage/2, B Voltage/2, C Voltage/2
  B Phase/1 -> B Sine/1
  B Sine/1 -> B Voltage/1
  C Phase/1 -> C Sine/1
  C Sine/1 -> C Voltage/1
  A Voltage/1 -> Three-Phase Voltage/1
  B Voltage/1 -> Three-Phase Voltage/2
  C Voltage/1 -> Three-Phase Voltage/3
  Vll_ref_V/1 -> Phase Peak/1
  enable/1 -> Enable Bounds/1
  Three-Phase Voltage/1 -> Apply Enable/1
  Enable Bounds/1 -> Apply Enable/2, enabled/1
  Apply Enable/1 -> vabc_V/1

== system bess_resource_standalone/BESS Resource/02 PCS/03 Virtual Impedance Interface/01 Current Conditioning ==
  iabc_A : Inport
  Clarke Current : Gain  Gain=sqrt(2/3)*[1 -0.5 -0.5;0 sqrt(3)/2 -sqrt(3)/2]  Multiplication=Matrix(K*u)
  Current Filter A : TransferFcn  Numerator=1  Denominator=[V2.BESS.control.virtual_impedance_measurement_tau_s 1]
  Current Filter B : TransferFcn  Numerator=1  Denominator=[V2.BESS.control.virtual_impedance_measurement_tau_s 1]
  Current Filter C : TransferFcn  Numerator=1  Denominator=[V2.BESS.control.virtual_impedance_measurement_tau_s 1]
  Filtered Current abc : Mux  Inputs=3
  Split Current : Demux  Outputs=3
  i_alpha_beta_A : Outport
  wires:
  iabc_A/1 -> Split Current/1
  Split Current/1 -> Current Filter A/1
  Current Filter A/1 -> Filtered Current abc/1
  Split Current/2 -> Current Filter B/1
  Current Filter B/1 -> Filtered Current abc/2
  Split Current/3 -> Current Filter C/1
  Current Filter C/1 -> Filtered Current abc/3
  Filtered Current abc/1 -> Clarke Current/1
  Clarke Current/1 -> i_alpha_beta_A/1

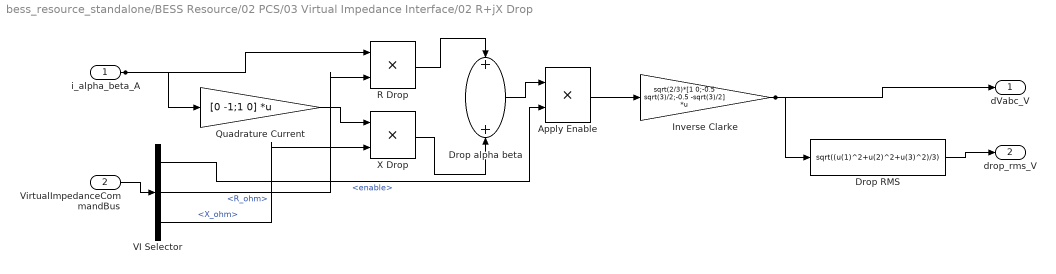
== system bess_resource_standalone/BESS Resource/02 PCS/03 Virtual Impedance Interface/02 R+jX Drop ==
  i_alpha_beta_A : Inport
  VirtualImpedanceCommandBus : Inport  Port=2  OutDataTypeStr=Bus: VirtualImpedanceCommandBus
  Apply Enable : Product
  Drop RMS : Fcn  Expr=sqrt((u(1)^2+u(2)^2+u(3)^2)/3)
  Drop alpha beta : Sum
  Inverse Clarke : Gain  Gain=sqrt(2/3)*[1 0;-0.5 sqrt(3)/2;-0.5 -sqrt(3)/2]  Multiplication=Matrix(K*u)
  Quadrature Current : Gain  Gain=[0 -1;1 0]  Multiplication=Matrix(K*u)
  R Drop : Product
  VI Selector : BusSelector  OutputSignals=enable,R_ohm,X_ohm
  X Drop : Product
  dVabc_V : Outport
  drop_rms_V : Outport  Port=2
  wires:
  VirtualImpedanceCommandBus/1 -> VI Selector/1
  i_alpha_beta_A/1 -> R Drop/1, Quadrature Current/1
  VI Selector/2 -> R Drop/2  "<R_ohm>"
  Quadrature Current/1 -> X Drop/1
  VI Selector/3 -> X Drop/2  "<X_ohm>"
  R Drop/1 -> Drop alpha beta/1
  X Drop/1 -> Drop alpha beta/2
  Drop alpha beta/1 -> Apply Enable/1
  VI Selector/1 -> Apply Enable/2  "<enable>"
  Apply Enable/1 -> Inverse Clarke/1
  Inverse Clarke/1 -> dVabc_V/1, Drop RMS/1
  Drop RMS/1 -> drop_rms_V/1

== system bess_resource_standalone/BESS Resource/02 PCS/03 Virtual Impedance Interface/03 Voltage Command Compensation ==
  GFMVoltageCommandBus : Inport  OutDataTypeStr=Bus: GFMVoltageCommandBus
  dVabc_V : Inport  Port=2
  Command Selector : BusSelector  OutputSignals=vabc_V,theta_rad,omega_rad_s,Vll_ref_V,enabled
  Compensated Command : BusCreator  Inputs=5  OutDataTypeStr=Bus: GFMVoltageCommandBus
  Compensated Voltage : Sum  Inputs=+-
  GFMVoltageCommandBus Out : Outport  OutDataTypeStr=Bus: GFMVoltageCommandBus
  wires:
  GFMVoltageCommandBus/1 -> Command Selector/1
  Command Selector/1 -> Compensated Voltage/1  "<vabc_V>"
  dVabc_V/1 -> Compensated Voltage/2
  Compensated Voltage/1 -> Compensated Command/1  "vabc_V"
  Command Selector/2 -> Compensated Command/2  "<theta_rad>"
  Command Selector/3 -> Compensated Command/3  "<omega_rad_s>"
  Command Selector/4 -> Compensated Command/4  "<Vll_ref_V>"
  Command Selector/5 -> Compensated Command/5  "<enabled>"
  Compensated Command/1 -> GFMVoltageCommandBus Out/1
